simulink model "ConvertidorDCDC_ControlObservador"  (R2026a)
settings: Solver=ode45  StopTime=1.5  MaxStep=1e-4  RelTol=1e-6
model workspace (MAT data in the model file):
  A = [0  -83.33; 500  -10]
  B = [166.67; 0]
  C = [0 1]
  K = [0.27599448011 -0.494115860381]
  Ke = 0.147767336739
  L = [-21.7590449644; 150]
  x0 = [2; 1]
  xh0 = [0; 0]
settings Model: Creator=jordy  LastModifiedBy=jordy

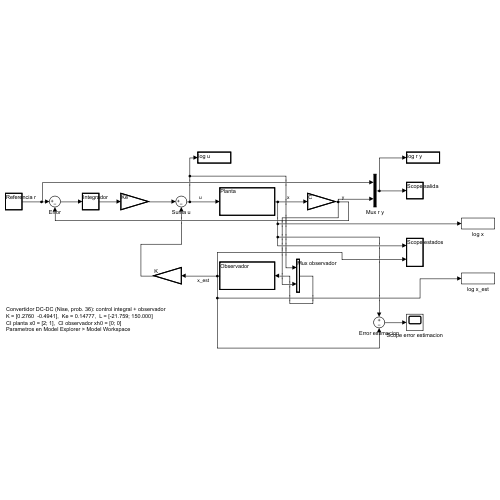
[thumbnail: Simulink's stored preview of the top-level diagram]
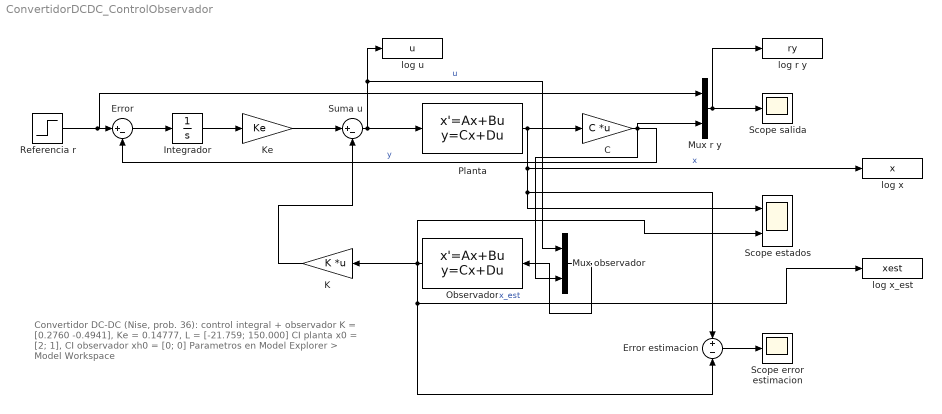
== system ConvertidorDCDC_ControlObservador ==
  note: Convertidor DC-DC (Nise, prob. 36): control integral + observador
      | K = [0.2760  -0.4941],  Ke = 0.14777,  L = [-21.759; 150.000]
      | CI planta x0 = [2; 1],  CI observador xh0 = [0; 0]
      | Parametros en Model Explorer > Model Workspace
  C : Gain  Gain=C  Multiplication=Matrix(K*u)
  Error : Sum  Inputs=|+-
  Error estimacion : Sum  Inputs=+-
  Integrador : Integrator
  K : Gain  Gain=K  Multiplication=Matrix(K*u)
  Ke : Gain  Gain=Ke
  Mux observador : Mux  Inputs=2
  Mux r y : Mux  Inputs=2
  Observador : StateSpace  A=A - L*C  B=[B L]  C=eye(2)  D=zeros(2,2)  InitialCondition=xh0
  Planta : StateSpace  A=A  B=B  C=eye(2)  D=zeros(2,1)  InitialCondition=x0
  Referencia r : Step  Time=0  SampleTime=0
  Scope error estimacion : Scope
  Scope estados : Scope  NumInputPorts=2
  Scope salida : Scope
  Suma u : Sum  Inputs=|+-
  log r y : ToWorkspace  VariableName=ry  SaveFormat=Timeseries  SampleTime=-1
  log u : ToWorkspace  VariableName=u  SaveFormat=Timeseries  SampleTime=-1
  log x : ToWorkspace  VariableName=x  SaveFormat=Timeseries  SampleTime=-1
  log x_est : ToWorkspace  VariableName=xest  SaveFormat=Timeseries  SampleTime=-1
  wires:
  Referencia r/1 -> Error/1, Mux r y/1
  Error/1 -> Integrador/1
  Integrador/1 -> Ke/1
  Ke/1 -> Suma u/1
  Suma u/1 -> Mux observador/1, log u/1, Planta/1  "u"
  Planta/1 -> Scope estados/1, Error estimacion/1, log x/1, C/1  "x"
  C/1 -> Error/2, Mux observador/2, Mux r y/2  "y"
  Mux r y/1 -> Scope salida/1, log r y/1
  Mux observador/1 -> Observador/1
  Observador/1 -> Error estimacion/2, log x_est/1, K/1, Scope estados/2  "x_est"
  K/1 -> Suma u/2
  Error estimacion/1 -> Scope error estimacion/1
